simulink model "Solar_EV_BESS_Full_Sys"  (R2024b)
settings: Solver=VariableStepAuto  StartTime=0.0  StopTime=1  RelTol=1e-3
libraries: spsSeriesRLCBranchLib x17, spsDiodeLib x15, spsPVArrayLib x12, spsVoltageMeasurementLib x6, spsCurrentMeasurementLib x5, spsIGBTDiodeLib x5, slpidlib x3, spsDCVoltageSourceLib x2, simulink x2, spspowerguiLib x1
settings Model: Creator=Bos we Tol  LastModifiedBy=Eng.Abd-Elrhman Saad
settings RTWCC: GPUComputeCapability=3.5

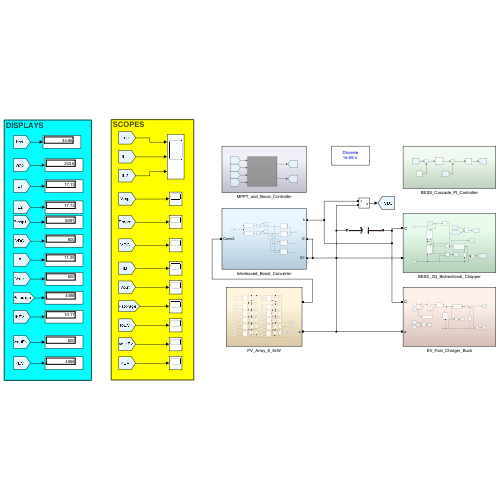
[thumbnail: Simulink's stored preview of the top-level diagram]
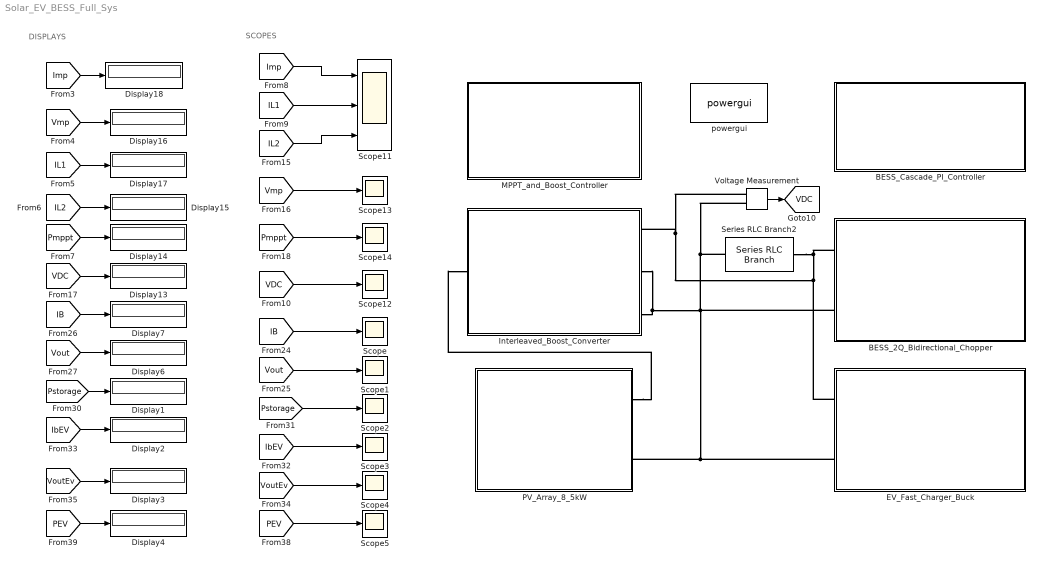
== system Solar_EV_BESS_Full_Sys ==
  note: SCOPES
  note: DISPLAYS
  BESS_2Q_Bidirectional_Chopper : Subsystem
  BESS_Cascade_PI_Controller : Subsystem
  Display{1..4,6..7,13..18} (12 alike) : Display
  EV_Fast_Charger_Buck : Subsystem
  Interleaved_Boost_Converter : Subsystem
  MPPT_and_Boost_Controller : Subsystem
  PV_Array_8_5kW : Subsystem
  Scope{,1..5,12..14} (9 alike) : Scope
  Scope11 : Scope  NumInputPorts=3
  Series RLC Branch2 : spsSeriesRLCBranchLib/Series RLC Branch  LConnTagsString=__new0  RConnTagsString=__new0  BranchType=C  Resistance=1  Inductance=1e-3  SetiL0=off  InitialCurrent=0  Capacitance=50e-03  Setx0=on  InitialVoltage=600  Measurements=None
  Voltage Measurement : spsVoltageMeasurementLib/Voltage Measurement  PhasorSimulation=off  OutputType=Complex  PSBequivalent=0
  powergui : spspowerguiLib/powergui  Priority=1  SimulationMode=Discrete  SampleTime=1e-06  frequency=60  Iterations=50  frequencyindice=0  Pbase=100e6  ErrMax=1e-4  UnitsV=kV  UnitsW=MW  buscounter=0  FunctionMessages=off  echomessages=off  EnableUseOfTLC=off  CurrentSourceSwitches=off  DisableSnubberDevices=off  DisableRonSwitches=off  DisableVfSwitches=off  DisplayEquations=off  AutomaticDiscreteSolvers=off  SolverType=Tustin/Backward Euler (TBE)  Interpol=off  ExternalGateDelay=off  methode=off  Ts=100  x0status=blocks  SPID=on  SwTol=0  HookPort=off  NonlinearTolerance=1e-4  nMaxIteration=100  ContinueOnMaxIteration=off  RestoreLinks=warning  ResistiveCurrentMeasurement=off  Frange=[0:2:500]  Ylog=off  Xlog=on  ShowGrid=off  save=off  variable=ZData  structure=0  ZoomFFT=off  StartTime=0.0  cycles=1  DisplayStyle=1  fundamental=60  FreqAxis=off  MaxFrequency=1000  frequencyindicesteady=1  RmsSteady=1  display=off
  tag scope: VDC=global
  wires:
  [Imp] -> Scope11/1
  [IL2] -> Display15/1
  [Pmppt] -> Display14/1
  [VDC] -> Display13/1
  [Vmp] -> Scope13/1
  [Pmppt] -> Scope14/1
  [IL1] -> Display17/1
  [Imp] -> Display18/1
  [IL2] -> Scope11/3
  [IL1] -> Scope11/2
  [VDC] -> Scope12/1
  [Vmp] -> Display16/1
  Voltage Measurement/1 -> [VDC]
  [IB] -> Scope/1
  [Vout] -> Scope1/1
  [IB] -> Display7/1
  [Vout] -> Display6/1
  [Pstorage] -> Display1/1
  [Pstorage] -> Scope2/1
  [IbEV] -> Scope3/1
  [IbEV] -> Display2/1
  [VoutEv] -> Scope4/1
  [VoutEv] -> Display3/1
  [PEV] -> Scope5/1
  [PEV] -> Display4/1
  connections:
  Voltage Measurement/LConn2 -- EV_Fast_Charger_Buck/LConn2 -- PV_Array_8_5kW/RConn2 -- BESS_2Q_Bidirectional_Chopper/LConn2 -- Interleaved_Boost_Converter/RConn2 -- Interleaved_Boost_Converter/RConn3 -- Series RLC Branch2/RConn1
  Series RLC Branch2/LConn1 -- BESS_2Q_Bidirectional_Chopper/LConn1 -- Voltage Measurement/LConn1 -- Interleaved_Boost_Converter/RConn1 -- EV_Fast_Charger_Buck/LConn1
  PV_Array_8_5kW/RConn1 -- Interleaved_Boost_Converter/LConn1

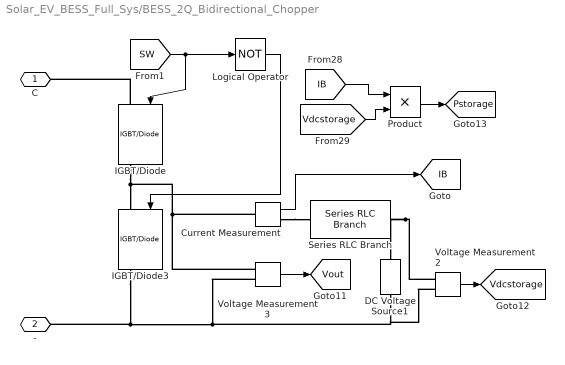
== system Solar_EV_BESS_Full_Sys/BESS_2Q_Bidirectional_Chopper ==
  Current Measurement : spsCurrentMeasurementLib/Current Measurement  PhasorSimulation=off  OutputType=Complex  PSBequivalent=0
  DC Voltage Source1 : spsDCVoltageSourceLib/DC Voltage Source  Amplitude=400  Measurements=None
  IGBT/Diode : spsIGBTDiodeLib/IGBT//Diode  Ron=1e-3  Rs=1e5  Cs=inf  Measurements=on
  IGBT/Diode3 : spsIGBTDiodeLib/IGBT//Diode  Ron=1e-3  Rs=1e5  Cs=inf  Measurements=on
  Logical Operator : Logic  Operator=NOT  AllPortsSameDT=off  OutDataTypeStr=boolean
  Product : Product
  Series RLC Branch : spsSeriesRLCBranchLib/Series RLC Branch  LConnTagsString=__new0  RConnTagsString=__new0  BranchType=L  Resistance=1  Inductance=30e-3  SetiL0=off  InitialCurrent=0  Capacitance=1e-6  Setx0=off  InitialVoltage=0  Measurements=None
  Voltage Measurement2 : spsVoltageMeasurementLib/Voltage Measurement  PhasorSimulation=off  OutputType=Complex  PSBequivalent=0
  Voltage Measurement3 : spsVoltageMeasurementLib/Voltage Measurement  PhasorSimulation=off  OutputType=Complex  PSBequivalent=0
  C : PMIOPort  Side=Left
  - : PMIOPort  Port=2  Side=Left
  tag scope: IB=global, Pstorage=global, Vdcstorage=global, Vout=global
  wires:
  [SW] -> IGBT/Diode/1, Logical Operator/1
  [Vdcstorage] -> Product/2
  Voltage Measurement3/1 -> [Vout]
  Logical Operator/1 -> IGBT/Diode3/1
  Product/1 -> [Pstorage]
  Voltage Measurement2/1 -> [Vdcstorage]
  Current Measurement/1 -> [IB]
  [IB] -> Product/1
  connections:
  IGBT/Diode3/RConn1 -- -/RConn1 -- Voltage Measurement2/LConn2 -- DC Voltage Source1/LConn1 -- Voltage Measurement3/LConn2
  Current Measurement/RConn1 -- Series RLC Branch/LConn1
  Series RLC Branch/RConn1 -- Voltage Measurement2/LConn1 -- DC Voltage Source1/RConn1
  Current Measurement/LConn1 -- Voltage Measurement3/LConn1 -- IGBT/Diode/RConn1 -- IGBT/Diode3/LConn1
  IGBT/Diode/LConn1 -- C/RConn1

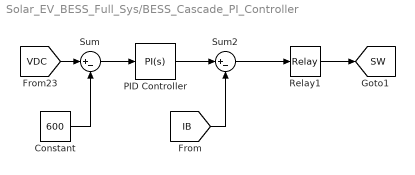
== system Solar_EV_BESS_Full_Sys/BESS_Cascade_PI_Controller ==
  Constant : Constant  Value=600
  PID Controller : slpidlib/PID Controller  Controller=PI  Form=Parallel  TimeDomain=Continuous-time  UseExternalTs=off  SampleTime=-1  IntegratorMethod=Forward Euler  FilterMethod=Forward Euler  ControllerParametersSource=internal  P=1  I=100  UseKiTs=off  D=0  UseExternalDerivativeSource=off  N=100  UseFilter=on  TunerSelectOption=Transfer Function Based (PID Tuner App)  InitialConditionSource=internal  InitialConditionForIntegrator=0  InitialConditionForFilter=0  DifferentiatorICPrevScaledInput=0  ExternalReset=none  TrackingMode=off  Kt=1  LimitOutput=off  SatLimitsSource=internal  UpperSaturationLimit=inf  LowerSaturationLimit=-inf  LinearizeAsGain=on  AntiWindupMode=none  Kb=1  LimitIntegrator=off  UpperIntegratorSaturationLimit=inf  LowerIntegratorSaturationLimit=-inf  POutMin=[]  POutMax=[]  IOutMin=[]  IOutMax=[]  DOutMin=[]  DOutMax=[]  NOutMin=[]  NOutMax=[]  SumOutMin=[]  SumOutMax=[]  SaturationOutMin=[]  SaturationOutMax=[]  PParamMin=[]  PParamMax=[]  IParamMin=[]  IParamMax=[]  DParamMin=[]  DParamMax=[]  NParamMin=[]  NParamMax=[]  KbParamMin=[]  KbParamMax=[]  KtParamMin=[]  KtParamMax=[]  KbOutMin=[]  KbOutMax=[]  KtOutMin=[]  KtOutMax=[]  IntegratorOutMin=[]  IntegratorOutMax=[]  FilterOutMin=[]  FilterOutMax=[]  SumI1OutMin=[]  SumI1OutMax=[]  SumI2OutMin=[]  SumI2OutMax=[]  SumI3OutMin=[]  SumI3OutMax=[]  SumI4OutMin=[]  SumI4OutMax=[]  SumDOutMin=[]  SumDOutMax=[]  DifferentiatorOutMin=[]  DifferentiatorOutMax=[]  FilterDiffOutCoefMin=[]  FilterDiffOutCoefMax=[]  ReciprocalOutMin=[]  ReciprocalOutMax=[]  SumDenOutMin=[]  SumDenOutMax=[]  SumNumOutMin=[]  SumNumOutMax=[]  DivideOutMin=[]  DivideOutMax=[]  UdiffTsProdOutMin=[]  UdiffTsProdOutMax=[]  NTsProdOutMin=[]  NTsProdOutMax=[]  UintegralTsProdOutMin=[]  UintegralTsProdOutMax=[]  UngainTsProdOutMin=[]  UngainTsProdOutMax=[]  ClampingZeroOutDataTypeStr=Inherit: Inherit via back propagation  ClampingZeroOutMin=[]  ClampingZeroOutMax=[]  FilterDenConstantOutDataTypeStr=Inherit: Inherit via back propagation  FilterDenConstantOutMin=[]  FilterDenConstantOutMax=[]  PCopyOutDataTypeStr=Inherit: Inherit via back propagation  PCopyOutMin=[]  PCopyOutMax=[]  NCopyOutDataTypeStr=Inherit: Inherit via back propagation  NCopyOutMin=[]  NCopyOutMax=[]  IntegratorContinuousStateAttributes=''  IntegratorStateMustResolveToSignalObject=off  IntegratorRTWStateStorageClass=Auto  FilterContinuousStateAttributes=''  FilterStateMustResolveToSignalObject=off  FilterRTWStateStorageClass=Auto  ParallelPVariant=InternalParameters  IdealPVariant=Disabled  IVariant=InternalParameters  DVariant=Disabled  IntegratorVariant=Continuous  SatVariant=Disabled  AWVariant=Passthrough  PCopyVariant=Disabled  TRVariant=Disabled  FdbkBlocksVariant=Forward  IdealPFdbkVariant=Disabled  SatFdbkVariant=Disabled  DerivativeFilterVariant=Disabled  NVariant=Disabled  NCopyVariant=Disabled_SignalSpec  FilterICVariant=Disabled  IntegratorICVariant=InternalICs  ExternalResetVariant=Disabled  TRSumVariant=Passthrough  SumFdbkVariant=Disabled  SumVariant=Sum_PI  TsampFilterVariant=InternalTs  TsampNgainVariant=Passthrough  TsampIntegralVariant=Disabled_SignalSpec  ExternalSaturationOutDataTypeStr=Inherit: Same as second input  DerivativeSourceVariant=Disabled  PreIntVariant=InternalPreInt
  Relay1 : Relay  OnSwitchValue=0.2  OffSwitchValue=-0.2
  Sum : Sum  Inputs=|+-
  Sum2 : Sum  Inputs=|+-
  tag scope: SW=global
  wires:
  Constant/1 -> Sum/2
  Relay1/1 -> [SW]
  Sum/1 -> PID Controller/1
  Sum2/1 -> Relay1/1
  [IB] -> Sum2/2
  [VDC] -> Sum/1
  PID Controller/1 -> Sum2/1

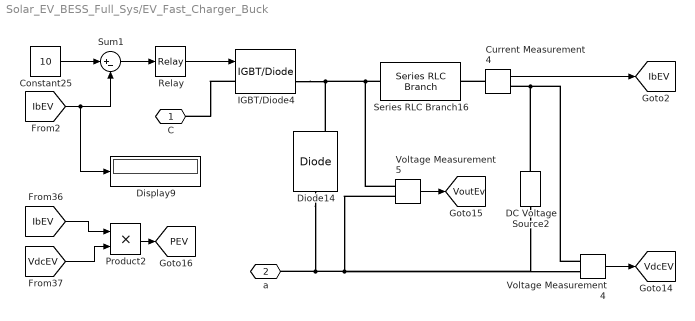
== system Solar_EV_BESS_Full_Sys/EV_Fast_Charger_Buck ==
  Constant25 : Constant  Value=10
  Current Measurement4 : spsCurrentMeasurementLib/Current Measurement  PhasorSimulation=off  OutputType=Complex  PSBequivalent=0
  DC Voltage Source2 : spsDCVoltageSourceLib/DC Voltage Source  Amplitude=400  Measurements=None
  Diode14 : spsDiodeLib/Diode  Ron=0.001  Lon=0  Vf=0  IC=0  UseSnubber=0  Rs=50000  Cs=250e-9  Measurements=on
  Display9 : Display
  IGBT/Diode4 : spsIGBTDiodeLib/IGBT//Diode  Ron=1e-3  Rs=1e5  Cs=inf  Measurements=on
  Product2 : Product
  Relay : Relay  OnSwitchValue=0.2  OffSwitchValue=-0.2
  Series RLC Branch16 : spsSeriesRLCBranchLib/Series RLC Branch  LConnTagsString=__new0  RConnTagsString=__new0  BranchType=L  Resistance=1  Inductance=30e-3  SetiL0=off  InitialCurrent=0  Capacitance=1e-6  Setx0=off  InitialVoltage=0  Measurements=None
  Sum1 : Sum  Inputs=|+-
  Voltage Measurement4 : spsVoltageMeasurementLib/Voltage Measurement  PhasorSimulation=off  OutputType=Complex  PSBequivalent=0
  Voltage Measurement5 : spsVoltageMeasurementLib/Voltage Measurement  PhasorSimulation=off  OutputType=Complex  PSBequivalent=0
  C : PMIOPort  Side=Left
  a : PMIOPort  Port=2  Side=Left
  tag scope: IbEV=global, PEV=global, VdcEV=global, VoutEv=global
  wires:
  [IbEV] -> Sum1/2, Display9/1
  Product2/1 -> [PEV]
  Sum1/1 -> Relay/1
  Relay/1 -> IGBT/Diode4/1
  Constant25/1 -> Sum1/1
  Voltage Measurement5/1 -> [VoutEv]
  Voltage Measurement4/1 -> [VdcEV]
  [IbEV] -> Product2/1
  [VdcEV] -> Product2/2
  Current Measurement4/1 -> [IbEV]
  connections:
  DC Voltage Source2/RConn1 -- Voltage Measurement4/LConn1 -- Current Measurement4/RConn1
  Voltage Measurement5/LConn2 -- Diode14/LConn1 -- a/RConn1 -- Voltage Measurement4/LConn2 -- DC Voltage Source2/LConn1
  Series RLC Branch16/LConn1 -- Diode14/RConn1 -- IGBT/Diode4/RConn1 -- Voltage Measurement5/LConn1
  Current Measurement4/LConn1 -- Series RLC Branch16/RConn1
  IGBT/Diode4/LConn1 -- C/RConn1

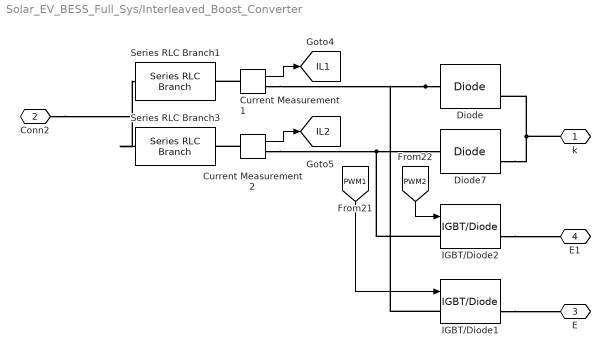
== system Solar_EV_BESS_Full_Sys/Interleaved_Boost_Converter ==
  Current Measurement1 : spsCurrentMeasurementLib/Current Measurement  PhasorSimulation=off  OutputType=Complex  PSBequivalent=0
  Current Measurement2 : spsCurrentMeasurementLib/Current Measurement  PhasorSimulation=off  OutputType=Complex  PSBequivalent=0
  Diode : spsDiodeLib/Diode  Ron=0.001  Lon=0  Vf=0.8  IC=0  UseSnubber=0  Rs=500000  Cs=250e-9  Measurements=on
  Diode7 : spsDiodeLib/Diode  Ron=0.001  Lon=0  Vf=0.8  IC=0  UseSnubber=0  Rs=500000  Cs=250e-9  Measurements=on
  IGBT/Diode1 : spsIGBTDiodeLib/IGBT//Diode  Ron=0.001  Rs=1e5  Cs=inf  Measurements=on
  IGBT/Diode2 : spsIGBTDiodeLib/IGBT//Diode  Ron=0.001  Rs=1e5  Cs=inf  Measurements=on
  Series RLC Branch1 : spsSeriesRLCBranchLib/Series RLC Branch  LConnTagsString=__new0  RConnTagsString=__new0  BranchType=L  Resistance=1  Inductance=20e-03  SetiL0=off  InitialCurrent=0  Capacitance=1e-6  Setx0=off  InitialVoltage=0  Measurements=None
  Series RLC Branch3 : spsSeriesRLCBranchLib/Series RLC Branch  LConnTagsString=__new0  RConnTagsString=__new0  BranchType=L  Resistance=1  Inductance=20e-03  SetiL0=off  InitialCurrent=0  Capacitance=1e-6  Setx0=off  InitialVoltage=0  Measurements=None
  k : PMIOPort  Side=Right
  Conn2 : PMIOPort  Port=2  Side=Left
  E : PMIOPort  Port=3  Side=Right
  E1 : PMIOPort  Port=4  Side=Right
  tag scope: IL1=global, IL2=global
  wires:
  [PWM2] -> IGBT/Diode2/1
  [PWM1] -> IGBT/Diode1/1
  Current Measurement1/1 -> [IL1]
  Current Measurement2/1 -> [IL2]
  connections:
  Diode7/RConn1 -- Diode/RConn1 -- k/RConn1
  Series RLC Branch3/LConn1 -- Conn2/RConn1 -- Series RLC Branch1/LConn1
  Current Measurement1/LConn1 -- Series RLC Branch1/RConn1
  Current Measurement2/RConn1 -- Diode7/LConn1 -- IGBT/Diode2/LConn1
  Diode/LConn1 -- Current Measurement1/RConn1 -- IGBT/Diode1/LConn1
  Current Measurement2/LConn1 -- Series RLC Branch3/RConn1
  IGBT/Diode2/RConn1 -- E1/RConn1
  IGBT/Diode1/RConn1 -- E/RConn1

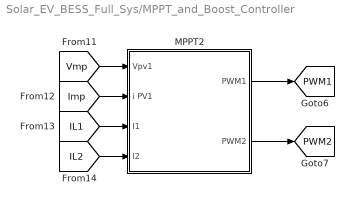
== system Solar_EV_BESS_Full_Sys/MPPT_and_Boost_Controller ==
  MPPT2 : Subsystem
  tag scope: PWM1=global, PWM2=global
  wires:
  MPPT2/1(PWM1) -> [PWM1]
  [Vmp] -> MPPT2/1(Vpv1)
  MPPT2/2(PWM2) -> [PWM2]
  [IL2] -> MPPT2/4(I2)
  [Imp] -> MPPT2/2(i PV1)
  [IL1] -> MPPT2/3(I1)

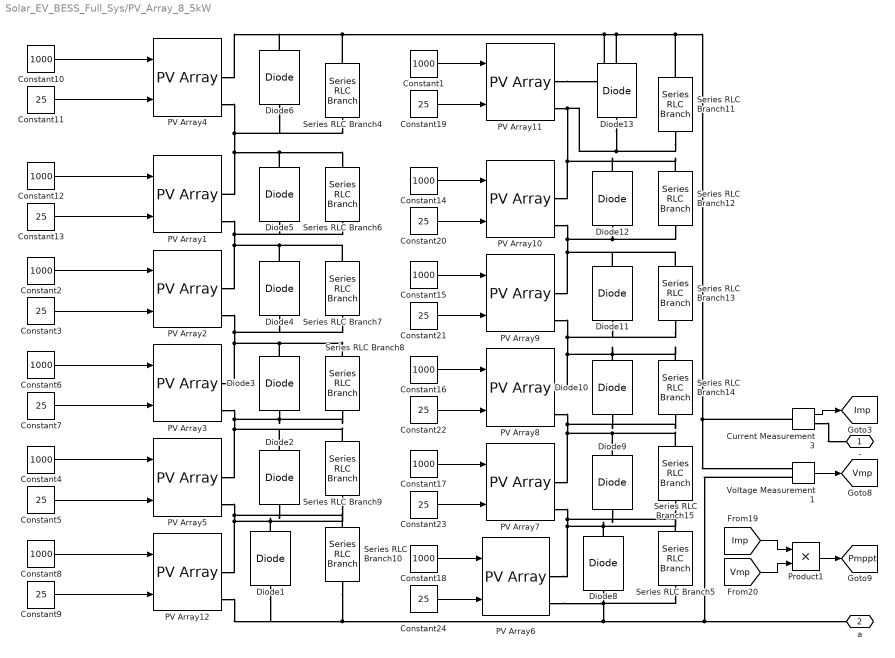
== system Solar_EV_BESS_Full_Sys/PV_Array_8_5kW ==
  Constant{1..2,4,6,8,10,12,14..18} (12 alike) : Constant  Value=1000
  Constant{3,5,7,9,11,13,19..24} (12 alike) : Constant  Value=25
  Current Measurement3 : spsCurrentMeasurementLib/Current Measurement  PhasorSimulation=off  OutputType=Complex  PSBequivalent=0
  Diode{1..6,8..13} (12 alike) : spsDiodeLib/Diode  Ron=0.001  Lon=0  Vf=0  IC=0  UseSnubber=0  Rs=50000  Cs=250e-9  Measurements=off
  PV Array{1..12} (12 alike) : spsPVArrayLib/PV Array  Npar=1  Nser=1  PlotType=array @ 25 deg.C & specified irradiances  S_vec="[ 1000  500  100 ]"  Temp_C_vec="[ 45 25  ]"  ModuleName=User-defined  PlotWhenSelected=off  Pm=710.024  Ncell=96  Voc=49  Isc=18.4  Vm=40.9  Im=17.36  beta_Voc_pc=-0.36099  alpha_Isc_pc=0.102  beta_Voc=-0.17689  alpha_Isc=0.018768  IL=18.4744  I0=6.8764e-10  nI=0.82775  Rsh=197.1327  Rs=0.11278  RobustModel=off  RobustCellTemperature=313.3991  BAL=on  Tc=1e-6  Tfilter=5e-5
  Product1 : Product
  Series RLC Branch{5..10,12..15} (10 alike) : spsSeriesRLCBranchLib/Series RLC Branch  LConnTagsString=__new0  RConnTagsString=__new0  BranchType=C  Resistance=30  Inductance=1e-3  SetiL0=off  InitialCurrent=0  Capacitance=10e-6  Setx0=off  InitialVoltage=60  Measurements=None
  Series RLC Branch11 : spsSeriesRLCBranchLib/Series RLC Branch  LConnTagsString=__new0  RConnTagsString=__new0  BranchType=C  Resistance=30  Inductance=1e-3  SetiL0=off  InitialCurrent=0  Capacitance=100e-6  Setx0=off  InitialVoltage=60  Measurements=None
  Series RLC Branch4 : spsSeriesRLCBranchLib/Series RLC Branch  LConnTagsString=__new0  RConnTagsString=__new0  BranchType=C  Resistance=30  Inductance=1e-3  SetiL0=off  InitialCurrent=0  Capacitance=100e-6  Setx0=off  InitialVoltage=60  Measurements=None
  Voltage Measurement1 : spsVoltageMeasurementLib/Voltage Measurement  PhasorSimulation=off  OutputType=Complex  PSBequivalent=0
  - : PMIOPort  Side=Right
  a : PMIOPort  Port=2  Side=Right
  tag scope: Imp=global, Pmppt=global, Vmp=global
  wires:
  Constant23/1 -> PV Array7/2
  Constant1/1 -> PV Array11/1
  Constant18/1 -> PV Array6/1
  Constant21/1 -> PV Array9/2
  Constant22/1 -> PV Array8/2
  Constant20/1 -> PV Array10/2
  Constant8/1 -> PV Array12/1
  Product1/1 -> [Pmppt]
  Constant4/1 -> PV Array5/1
  Constant17/1 -> PV Array7/1
  Constant16/1 -> PV Array8/1
  Constant19/1 -> PV Array11/2
  Constant7/1 -> PV Array3/2
  [Vmp] -> Product1/2
  Constant11/1 -> PV Array4/2
  Constant13/1 -> PV Array1/2
  Constant6/1 -> PV Array3/1
  Current Measurement3/1 -> [Imp]
  Constant15/1 -> PV Array9/1
  Constant2/1 -> PV Array2/1
  Constant14/1 -> PV Array10/1
  Constant3/1 -> PV Array2/2
  Constant24/1 -> PV Array6/2
  Constant9/1 -> PV Array12/2
  Constant10/1 -> PV Array4/1
  Voltage Measurement1/1 -> [Vmp]
  Constant12/1 -> PV Array1/1
  [Imp] -> Product1/1
  Constant5/1 -> PV Array5/2
  connections:
  Series RLC Branch5/LConn1 -- Diode8/RConn1 -- PV Array6/RConn1 -- PV Array7/RConn2 -- Diode9/LConn1 -- Series RLC Branch15/RConn1
  Series RLC Branch11/LConn1 -- PV Array11/RConn1 -- Series RLC Branch4/LConn1 -- Diode6/RConn1 -- PV Array4/RConn1 -- Diode13/RConn1 -- Voltage Measurement1/LConn1 -- Current Measurement3/LConn1
  Diode1/RConn1 -- Series RLC Branch10/LConn1 -- PV Array12/RConn1 -- PV Array5/RConn2 -- Diode2/LConn1 -- Series RLC Branch9/RConn1
  Series RLC Branch11/RConn1 -- Diode13/LConn1 -- PV Array11/RConn2 -- Series RLC Branch12/LConn1 -- Diode12/RConn1 -- PV Array10/RConn1
  Diode3/RConn1 -- Series RLC Branch8/LConn1 -- PV Array3/RConn1 -- PV Array2/RConn2 -- Diode4/LConn1 -- Series RLC Branch7/RConn1
  Diode10/RConn1 -- Series RLC Branch14/LConn1 -- PV Array8/RConn1 -- PV Array9/RConn2 -- Diode11/LConn1 -- Series RLC Branch13/RConn1
  Diode4/RConn1 -- Series RLC Branch7/LConn1 -- PV Array2/RConn1 -- PV Array1/RConn2 -- Series RLC Branch6/RConn1 -- Diode5/LConn1
  PV Array6/RConn2 -- Series RLC Branch10/RConn1 -- Diode1/LConn1 -- PV Array12/RConn2 -- Voltage Measurement1/LConn2 -- a/RConn1 -- Series RLC Branch5/RConn1 -- Diode8/LConn1
  Series RLC Branch4/RConn1 -- Diode6/LConn1 -- PV Array4/RConn2 -- PV Array1/RConn1 -- Diode5/RConn1 -- Series RLC Branch6/LConn1
  Series RLC Branch12/RConn1 -- Diode12/LConn1 -- PV Array10/RConn2 -- PV Array9/RConn1 -- Series RLC Branch13/LConn1 -- Diode11/RConn1
  Diode3/LConn1 -- PV Array3/RConn2 -- PV Array5/RConn1 -- Diode2/RConn1 -- Series RLC Branch9/LConn1 -- Series RLC Branch8/RConn1
  Diode9/RConn1 -- Series RLC Branch15/LConn1 -- PV Array7/RConn1 -- PV Array8/RConn2 -- Diode10/LConn1 -- Series RLC Branch14/RConn1
  Current Measurement3/RConn1 -- -/RConn1

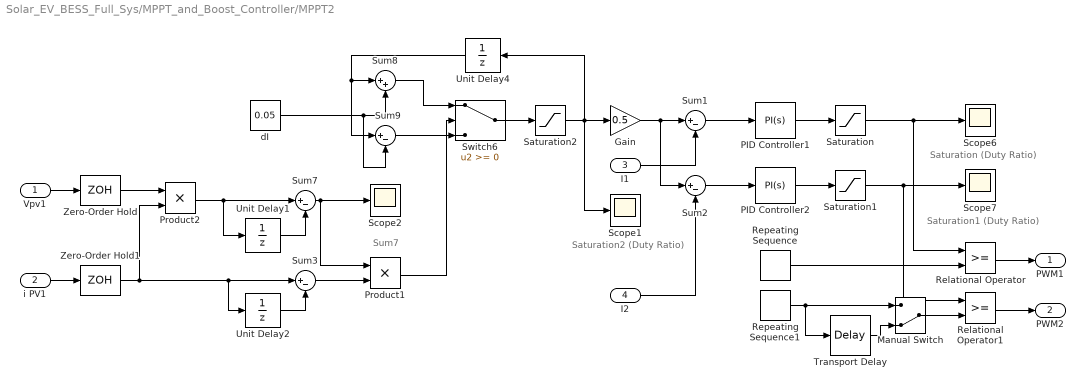
== system Solar_EV_BESS_Full_Sys/MPPT_and_Boost_Controller/MPPT2 ==
  note: Saturation2 (Duty Ratio)
  note: Sum7
  note: Saturation (Duty Ratio)
  note: Saturation1 (Duty Ratio)
  Vpv1 : Inport
  i PV1 : Inport  Port=2
  I1 : Inport  Port=3
  I2 : Inport  Port=4
  Gain : Gain  Gain=0.5
  Manual Switch : ManualSwitch  CurrentSetting=0
  PID Controller1 : slpidlib/PID Controller  Controller=PI  Form=Parallel  TimeDomain=Continuous-time  UseExternalTs=off  SampleTime=-1  IntegratorMethod=Forward Euler  FilterMethod=Forward Euler  ControllerParametersSource=internal  P=0.1  I=1  UseKiTs=off  D=0  UseExternalDerivativeSource=off  N=100  UseFilter=on  TunerSelectOption=Transfer Function Based (PID Tuner App)  InitialConditionSource=internal  InitialConditionForIntegrator=0  InitialConditionForFilter=0  DifferentiatorICPrevScaledInput=0  ExternalReset=none  TrackingMode=off  Kt=1  LimitOutput=off  SatLimitsSource=internal  UpperSaturationLimit=inf  LowerSaturationLimit=-inf  LinearizeAsGain=on  AntiWindupMode=none  Kb=1  LimitIntegrator=off  UpperIntegratorSaturationLimit=inf  LowerIntegratorSaturationLimit=-inf  POutMin=[]  POutMax=[]  IOutMin=[]  IOutMax=[]  DOutMin=[]  DOutMax=[]  NOutMin=[]  NOutMax=[]  SumOutMin=[]  SumOutMax=[]  SaturationOutMin=[]  SaturationOutMax=[]  PParamMin=[]  PParamMax=[]  IParamMin=[]  IParamMax=[]  DParamMin=[]  DParamMax=[]  NParamMin=[]  NParamMax=[]  KbParamMin=[]  KbParamMax=[]  KtParamMin=[]  KtParamMax=[]  KbOutMin=[]  KbOutMax=[]  KtOutMin=[]  KtOutMax=[]  IntegratorOutMin=[]  IntegratorOutMax=[]  FilterOutMin=[]  FilterOutMax=[]  SumI1OutMin=[]  SumI1OutMax=[]  SumI2OutMin=[]  SumI2OutMax=[]  SumI3OutMin=[]  SumI3OutMax=[]  SumI4OutMin=[]  SumI4OutMax=[]  SumDOutMin=[]  SumDOutMax=[]  DifferentiatorOutMin=[]  DifferentiatorOutMax=[]  FilterDiffOutCoefMin=[]  FilterDiffOutCoefMax=[]  ReciprocalOutMin=[]  ReciprocalOutMax=[]  SumDenOutMin=[]  SumDenOutMax=[]  SumNumOutMin=[]  SumNumOutMax=[]  DivideOutMin=[]  DivideOutMax=[]  UdiffTsProdOutMin=[]  UdiffTsProdOutMax=[]  NTsProdOutMin=[]  NTsProdOutMax=[]  UintegralTsProdOutMin=[]  UintegralTsProdOutMax=[]  UngainTsProdOutMin=[]  UngainTsProdOutMax=[]  ClampingZeroOutDataTypeStr=Inherit: Inherit via back propagation  ClampingZeroOutMin=[]  ClampingZeroOutMax=[]  FilterDenConstantOutDataTypeStr=Inherit: Inherit via back propagation  FilterDenConstantOutMin=[]  FilterDenConstantOutMax=[]  PCopyOutDataTypeStr=Inherit: Inherit via back propagation  PCopyOutMin=[]  PCopyOutMax=[]  NCopyOutDataTypeStr=Inherit: Inherit via back propagation  NCopyOutMin=[]  NCopyOutMax=[]  IntegratorContinuousStateAttributes=''  IntegratorStateMustResolveToSignalObject=off  IntegratorRTWStateStorageClass=Auto  FilterContinuousStateAttributes=''  FilterStateMustResolveToSignalObject=off  FilterRTWStateStorageClass=Auto  ParallelPVariant=InternalParameters  IdealPVariant=Disabled  IVariant=InternalParameters  DVariant=Disabled  IntegratorVariant=Continuous  SatVariant=Disabled  AWVariant=Passthrough  PCopyVariant=Disabled  TRVariant=Disabled  FdbkBlocksVariant=Forward  IdealPFdbkVariant=Disabled  SatFdbkVariant=Disabled  DerivativeFilterVariant=Disabled  NVariant=Disabled  NCopyVariant=Disabled_SignalSpec  FilterICVariant=Disabled  IntegratorICVariant=InternalICs  ExternalResetVariant=Disabled  TRSumVariant=Passthrough  SumFdbkVariant=Disabled  SumVariant=Sum_PI  TsampFilterVariant=InternalTs  TsampNgainVariant=Passthrough  TsampIntegralVariant=Disabled_SignalSpec  ExternalSaturationOutDataTypeStr=Inherit: Same as second input  DerivativeSourceVariant=Disabled  PreIntVariant=InternalPreInt
  PID Controller2 : slpidlib/PID Controller  Controller=PI  Form=Parallel  TimeDomain=Continuous-time  UseExternalTs=off  SampleTime=-1  IntegratorMethod=Forward Euler  FilterMethod=Forward Euler  ControllerParametersSource=internal  P=0.1  I=1  UseKiTs=off  D=0  UseExternalDerivativeSource=off  N=100  UseFilter=on  TunerSelectOption=Transfer Function Based (PID Tuner App)  InitialConditionSource=internal  InitialConditionForIntegrator=0  InitialConditionForFilter=0  DifferentiatorICPrevScaledInput=0  ExternalReset=none  TrackingMode=off  Kt=1  LimitOutput=off  SatLimitsSource=internal  UpperSaturationLimit=inf  LowerSaturationLimit=-inf  LinearizeAsGain=on  AntiWindupMode=none  Kb=1  LimitIntegrator=off  UpperIntegratorSaturationLimit=inf  LowerIntegratorSaturationLimit=-inf  POutMin=[]  POutMax=[]  IOutMin=[]  IOutMax=[]  DOutMin=[]  DOutMax=[]  NOutMin=[]  NOutMax=[]  SumOutMin=[]  SumOutMax=[]  SaturationOutMin=[]  SaturationOutMax=[]  PParamMin=[]  PParamMax=[]  IParamMin=[]  IParamMax=[]  DParamMin=[]  DParamMax=[]  NParamMin=[]  NParamMax=[]  KbParamMin=[]  KbParamMax=[]  KtParamMin=[]  KtParamMax=[]  KbOutMin=[]  KbOutMax=[]  KtOutMin=[]  KtOutMax=[]  IntegratorOutMin=[]  IntegratorOutMax=[]  FilterOutMin=[]  FilterOutMax=[]  SumI1OutMin=[]  SumI1OutMax=[]  SumI2OutMin=[]  SumI2OutMax=[]  SumI3OutMin=[]  SumI3OutMax=[]  SumI4OutMin=[]  SumI4OutMax=[]  SumDOutMin=[]  SumDOutMax=[]  DifferentiatorOutMin=[]  DifferentiatorOutMax=[]  FilterDiffOutCoefMin=[]  FilterDiffOutCoefMax=[]  ReciprocalOutMin=[]  ReciprocalOutMax=[]  SumDenOutMin=[]  SumDenOutMax=[]  SumNumOutMin=[]  SumNumOutMax=[]  DivideOutMin=[]  DivideOutMax=[]  UdiffTsProdOutMin=[]  UdiffTsProdOutMax=[]  NTsProdOutMin=[]  NTsProdOutMax=[]  UintegralTsProdOutMin=[]  UintegralTsProdOutMax=[]  UngainTsProdOutMin=[]  UngainTsProdOutMax=[]  ClampingZeroOutDataTypeStr=Inherit: Inherit via back propagation  ClampingZeroOutMin=[]  ClampingZeroOutMax=[]  FilterDenConstantOutDataTypeStr=Inherit: Inherit via back propagation  FilterDenConstantOutMin=[]  FilterDenConstantOutMax=[]  PCopyOutDataTypeStr=Inherit: Inherit via back propagation  PCopyOutMin=[]  PCopyOutMax=[]  NCopyOutDataTypeStr=Inherit: Inherit via back propagation  NCopyOutMin=[]  NCopyOutMax=[]  IntegratorContinuousStateAttributes=''  IntegratorStateMustResolveToSignalObject=off  IntegratorRTWStateStorageClass=Auto  FilterContinuousStateAttributes=''  FilterStateMustResolveToSignalObject=off  FilterRTWStateStorageClass=Auto  ParallelPVariant=InternalParameters  IdealPVariant=Disabled  IVariant=InternalParameters  DVariant=Disabled  IntegratorVariant=Continuous  SatVariant=Disabled  AWVariant=Passthrough  PCopyVariant=Disabled  TRVariant=Disabled  FdbkBlocksVariant=Forward  IdealPFdbkVariant=Disabled  SatFdbkVariant=Disabled  DerivativeFilterVariant=Disabled  NVariant=Disabled  NCopyVariant=Disabled_SignalSpec  FilterICVariant=Disabled  IntegratorICVariant=InternalICs  ExternalResetVariant=Disabled  TRSumVariant=Passthrough  SumFdbkVariant=Disabled  SumVariant=Sum_PI  TsampFilterVariant=InternalTs  TsampNgainVariant=Passthrough  TsampIntegralVariant=Disabled_SignalSpec  ExternalSaturationOutDataTypeStr=Inherit: Same as second input  DerivativeSourceVariant=Disabled  PreIntVariant=InternalPreInt
  Product1 : Product
  Product2 : Product
  Relational Operator : RelationalOperator  OutDataTypeStr=boolean  RndMeth=Simplest  InputSameDT=off
  Relational Operator1 : RelationalOperator  OutDataTypeStr=boolean  RndMeth=Simplest  InputSameDT=off
  Repeating Sequence : simulink/Sources/Repeating Sequence  rep_seq_t=[0 1/10000]  rep_seq_y=[0 1]
  Repeating Sequence1 : simulink/Sources/Repeating Sequence  rep_seq_t=[0 1/10000]  rep_seq_y=[0 1]
  Saturation : Saturate  UpperLimit=1  LowerLimit=0
  Saturation1 : Saturate  UpperLimit=1  LowerLimit=0
  Saturation2 : Saturate  UpperLimit=36  LowerLimit=10
  Scope{1..2,6..7} (4 alike) : Scope
  Sum{1..3,7,9} (5 alike) : Sum  Inputs=|+-
  Sum8 : Sum  Inputs=|++
  Switch6 : Switch  SaturateOnIntegerOverflow=off  InputSameDT=off
  Transport Delay : TransportDelay  DelayTime=1/10000/2
  Unit Delay1 : UnitDelay  SampleTime=-1  HasFrameUpgradeWarning=on
  Unit Delay2 : UnitDelay  SampleTime=-1  HasFrameUpgradeWarning=on
  Unit Delay4 : UnitDelay  InitialCondition=10  SampleTime=-1  HasFrameUpgradeWarning=on
  Zero-Order Hold : ZeroOrderHold  SampleTime=0.0002
  Zero-Order Hold1 : ZeroOrderHold  SampleTime=0.0002
  dI : Constant  Value=0.05
  PWM1 : Outport
  PWM2 : Outport  Port=2
  wires:
  Sum3/1 -> Product1/2
  i PV1/1 -> Zero-Order Hold1/1
  PID Controller1/1 -> Saturation/1
  Vpv1/1 -> Zero-Order Hold/1
  Unit Delay1/1 -> Sum7/2
  Unit Delay2/1 -> Sum3/2
  Zero-Order Hold/1 -> Product2/1
  Sum2/1 -> PID Controller2/1
  Sum8/1 -> Switch6/1
  Zero-Order Hold1/1 -> Product2/2, Unit Delay2/1, Sum3/1
  Product2/1 -> Sum7/1, Unit Delay1/1
  Unit Delay4/1 -> Sum9/1, Sum8/1
  dI/1 -> Sum8/2, Sum9/2
  Transport Delay/1 -> Manual Switch/2
  Sum7/1 -> Product1/1, Scope2/1
  Sum9/1 -> Switch6/3
  Product1/1 -> Switch6/2
  Switch6/1 -> Saturation2/1
  Saturation2/1 -> Gain/1, Scope1/1, Unit Delay4/1
  Saturation1/1 -> Scope7/1, Relational Operator1/1
  Gain/1 -> Sum1/1, Sum2/1
  I1/1 -> Sum1/2
  Saturation/1 -> Scope6/1, Relational Operator/1
  I2/1 -> Sum2/2
  Sum1/1 -> PID Controller1/1
  PID Controller2/1 -> Saturation1/1
  Repeating Sequence1/1 -> Manual Switch/1, Transport Delay/1
  Repeating Sequence/1 -> Relational Operator/2
  Manual Switch/1 -> Relational Operator1/2
  Relational Operator/1 -> PWM1/1
  Relational Operator1/1 -> PWM2/1
